simulink model "imu_complementaryfilter"  (R2025a)
settings: Solver=FixedStepAuto  StartTime=t0  StopTime=t_end  FixedStep=1/50  RelTol=1e-3
undefined symbols (not defined in the file or in its folder): alpha, dt, q0
settings Model: Creator=eoencue1  LastModifiedBy=eoencue1
settings DebuggingCC: SignalRangeChecking=warning

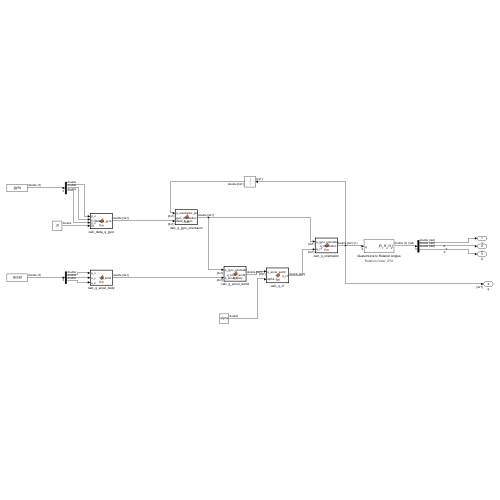
[thumbnail: Simulink's stored preview of the top-level diagram]
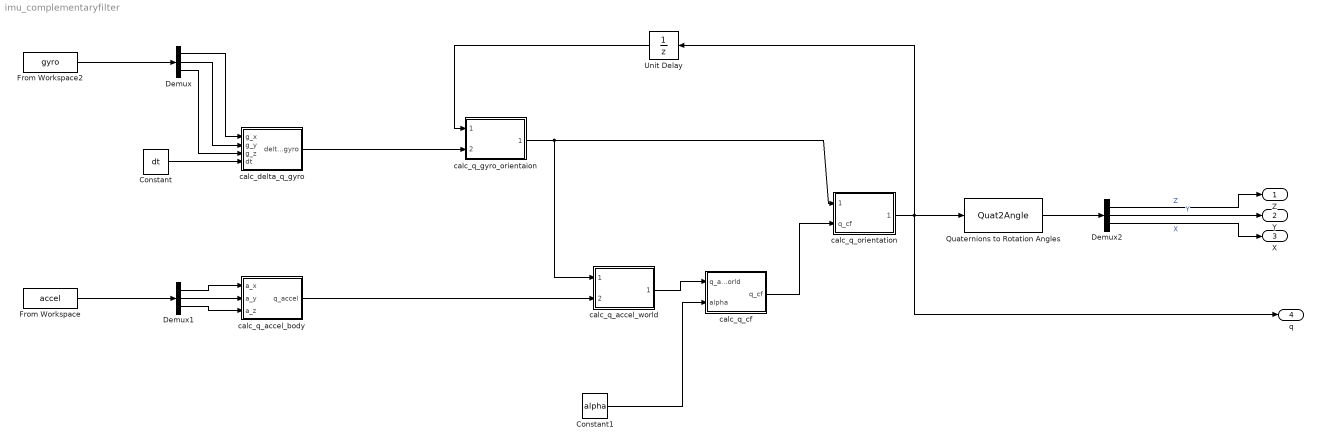
== system imu_complementaryfilter ==
  Constant : Constant  Value=dt
  Constant1 : Constant  Value=alpha
  Demux : Demux  Outputs=3
  Demux1 : Demux  Outputs=3
  Demux2 : Demux  Outputs=3
  From Workspace : FromWorkspace  VariableName=accel  SampleTime=1/50
  From Workspace2 : FromWorkspace  VariableName=gyro  SampleTime=1/50
  Quaternions to Rotation Angles : Quat2Angle
      settings: AttributesFormatString=Rotation Order: %<rotationOrder>
  Unit Delay : UnitDelay  InitialCondition=q0  SampleTime=-1  HasFrameUpgradeWarning=on
  calc_delta_q_gyro : MATLAB Function  TreatAsAtomicUnit=on
  calc_q_accel_body : MATLAB Function  TreatAsAtomicUnit=on
  calc_q_accel_world : MATLAB Function  TreatAsAtomicUnit=on
  calc_q_cf : MATLAB Function  TreatAsAtomicUnit=on
  calc_q_gyro_orientaion : MATLAB Function  TreatAsAtomicUnit=on
  calc_q_orientation : MATLAB Function  TreatAsAtomicUnit=on
  Z : Outport
  Y : Outport  Port=2
  X : Outport  Port=3
  q : Outport  Port=4
  wires:
  Constant/1 -> calc_delta_q_gyro/4(dt)
  Demux/1 -> calc_delta_q_gyro/1(g_x)
  Demux/2 -> calc_delta_q_gyro/2(g_y)
  Demux/3 -> calc_delta_q_gyro/3(g_z)
  From Workspace2/1 -> Demux/1
  calc_delta_q_gyro/1(delta_q_gyro) -> calc_q_gyro_orientaion/2(delta_q_gyro)
  From Workspace/1 -> Demux1/1
  Demux1/1 -> calc_q_accel_body/1(a_x)
  Demux1/2 -> calc_q_accel_body/2(a_y)
  Demux1/3 -> calc_q_accel_body/3(a_z)
  calc_q_accel_body/1(q_accel) -> calc_q_accel_world/2(q_accel_body)
  Unit Delay/1 -> calc_q_gyro_orientaion/1(q_orientation_prev)
  calc_q_gyro_orientaion/1(q_gyro_orientation) -> calc_q_accel_world/1(q_gyro_orientation), calc_q_orientation/1(q_gyro_orientaion)
  calc_q_cf/1(q_cf) -> calc_q_orientation/2(q_cf)
  calc_q_accel_world/1(q_accel_world) -> calc_q_cf/1(q_accel_world)
  calc_q_orientation/1(q_orientation) -> q/1, Quaternions to Rotation Angles/1, Unit Delay/1
  Constant1/1 -> calc_q_cf/2(alpha)
  Demux2/1 -> Z/1  "Z"
  Demux2/2 -> Y/1  "Y"
  Demux2/3 -> X/1  "X"
  Quaternions to Rotation Angles/1 -> Demux2/1

== matlab function imu_complementaryfilter/calc_q_gyro_orientaion ==
  data: q_orientation_prev input; delta_q_gyro input; q_gyro_orientation output
function q_gyro_orientation = fcn( q_orientation_prev,delta_q_gyro)

q_gyro_orientation = quaternion_mult(q_orientation_prev,delta_q_gyro);

== matlab function imu_complementaryfilter/calc_delta_q_gyro ==
  data: g_x input; delta_q_gyro output; g_y input; g_z input; dt input
function delta_q_gyro = fcn(g_x, g_y, g_z, dt)

w_betrag = sqrt(g_x^2+g_y^2+g_z^2);

if w_betrag < 1e-9
    delta_q_gyro = [1; 0; 0; 0];
    return;
end

w_x = g_x/w_betrag;
w_y = g_y/w_betrag;
w_z = g_z/w_betrag;

theta = w_betrag*dt;

delta_q_gyro =[cos(theta/2) ; w_x*sin(theta/2) ; w_y*sin(theta/2) ; w_z*sin(theta/2)];

== matlab function imu_complementaryfilter/calc_q_accel_body ==
  data: a_x input; q_accel output; a_y input; a_z input
function q_accel = fcn(a_x, a_y, a_z)

q_accel = [0 ; a_x ; a_y ;a_z];

== matlab function imu_complementaryfilter/calc_q_accel_world ==
  data: q_gyro_orientation input; q_accel_body input; q_accel_world output
function q_accel_world = fcn(q_gyro_orientation, q_accel_body)

q_gyro_orientation_inverse = [q_gyro_orientation(1) ; -q_gyro_orientation(2) ; -q_gyro_orientation(3) ; -q_gyro_orientation(4)];

q_gyro_accel = quaternion_mult(q_gyro_orientation,q_accel_body);

q_accel_world = quaternion_mult(q_gyro_accel,q_gyro_orientation_inverse);

== matlab function imu_complementaryfilter/calc_q_orientation ==
  data: q_gyro_orientaion input; q_orientation output; q_cf input
function q_orientation = fcn(q_gyro_orientaion, q_cf)

q_orientation = quaternion_mult(q_cf,q_gyro_orientaion);

== matlab function imu_complementaryfilter/calc_q_cf ==
  data: q_accel_world input; q_cf output; alpha input
function q_cf = fcn(q_accel_world, alpha)

q_accel_world_betrag = norm(q_accel_world);

phi = (1-alpha)*acos(q_accel_world(4)/q_accel_world_betrag);

v = [q_accel_world(2)/q_accel_world_betrag; q_accel_world(3)/q_accel_world_betrag ; q_accel_world(4)/q_accel_world_betrag];

n =  cross(v ,[0 ; 0 ; 1]);
n_betrag = norm(n);

q_cf = [cos(phi/2) ; (n(1)/n_betrag)*sin(phi/2) ; (n(2)/n_betrag)*sin(phi/2) ; (n(3)/n_betrag)*sin(phi/2)];
